simulink model "x280_canfd_loopback"  (R2024b)
settings: Solver=FixedStepDiscrete  StartTime=0.0  StopTime=inf  FixedStep=0.001  RelTol=1e-3
PreLoadFcn:
  | setupX280CANLibrary;
InitFcn:
  | setupX280CANLibrary;
libraries: x280_can_library x5, canfdmsglib x4
settings Model: Creator=Administrator  LastModifiedBy=Administrator
settings OptimizationCC: EnhancedBackFolding=on  PassReuseOutputArgsAs=Individual arguments  ZeroExternalMemoryAtStartup=off  ZeroInternalMemoryAtStartup=off  MaxStackSize=64  OptimizeBlockOrder=speed  DifferentSizesBufferReuse=on  OptimizationCustomize=off  EfficientTunableParamExpr=on
settings DebuggingCC: ParameterTunabilityLossMsg=error
settings HardwareCC: ProdBitPerLong=64  ProdHWDeviceType=Intel->x86-64 (Linux 64)
settings SFSimCC: MATLABDynamicMemAlloc=off
settings RTWCC: Description=Embedded Coder  SystemTargetFile=ert.tlc  HardwareBoard=SimRT  TLCOptions="-aInlineSetEventsForThisBaseRateFcn=TLC_FALSE -aSuppressMultiTaskScheduler=TLC_FALSE  -aRateBasedStepFcn=0"  TemplateMakefile=ert_default_tmf  Toolchain=X280 portable-linux-toolchain
settings CodeAppCC: ForceParamTrailComments=on  IgnoreCustomStorageClasses=off  OperatorAnnotations=on  SimulinkDataObjDesc=on  SFDataObjDesc=on  InsertBlockDesc=on
settings ERTTargetCC: ExtMode=on  ExtModeTransport=2  ExtModeStaticAlloc=on  ExtModeMexFile=ext_xcp  ExtModeIntrfLevel=Level2 - Open  InlinedParameterPlacement=Hierarchical

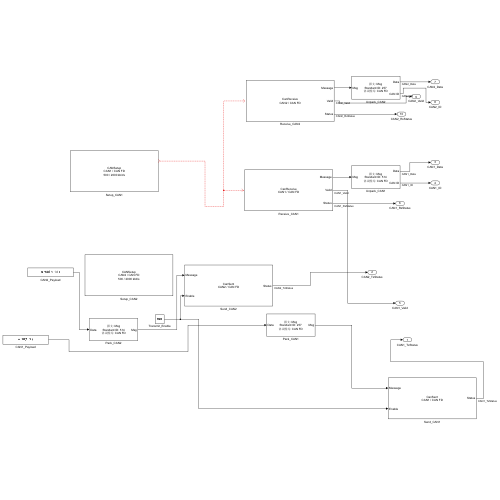
[thumbnail: Simulink's stored preview of the top-level diagram]
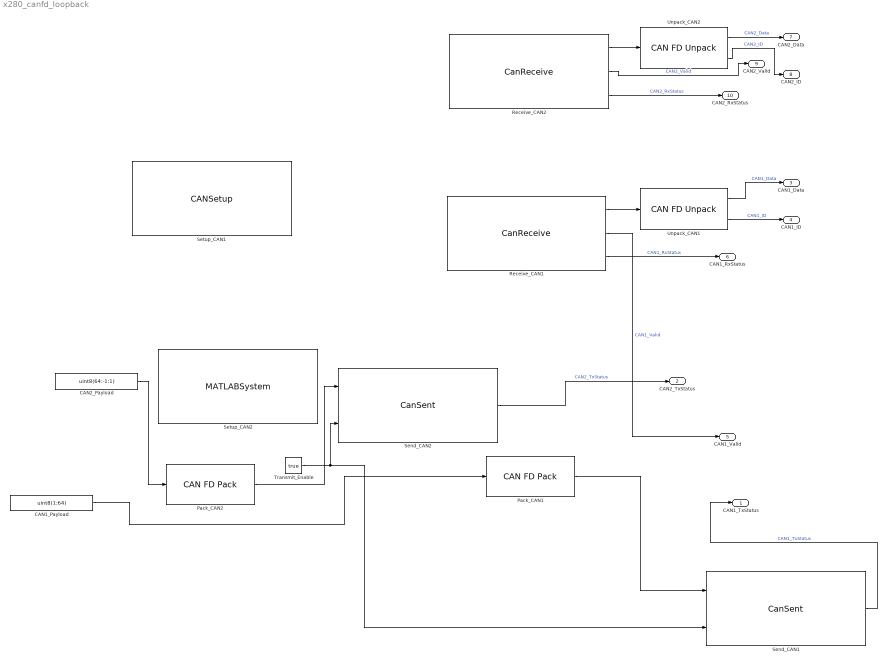
== system x280_canfd_loopback ==
  CAN1_Payload : Constant  Value=uint8(1:64)  SampleTime=0.001
  CAN2_Payload : Constant  Value=uint8(64:-1:1)  SampleTime=0.001
  Pack_CAN1 : canfdmsglib/CAN FD Pack  MsgList=(none)  MsgName=Msg  ProtocolMode=CAN FD  MsgIDType=Standard (11-bit identifier)  MsgIdentifier=257  CANIDInput=off  MsgLength=64  Remote=off  BRSSwitch=on  ApplyMinMax=off  SignalInfo={}
      settings: LibrarySourceBlock=canfdlib/CAN FD Pack  DataFormat=raw data
  Pack_CAN2 : canfdmsglib/CAN FD Pack  MsgList=(none)  MsgName=Msg  ProtocolMode=CAN FD  MsgIDType=Standard (11-bit identifier)  MsgIdentifier=514  CANIDInput=off  MsgLength=64  Remote=off  BRSSwitch=on  ApplyMinMax=off  SignalInfo={}
      settings: LibrarySourceBlock=canfdlib/CAN FD Pack  DataFormat=raw data
  Receive_CAN1 : x280_can_library/CanReceive  Priority=0  Channel=1  CANType=CAN FD  SampleTime=0.001
      settings: SourceProductName=X280 Linux TC1013 CAN
  Receive_CAN2 : x280_can_library/CanReceive  Priority=1  Channel=2  CANType=CAN FD  SampleTime=0.001
      settings: SourceProductName=X280 Linux TC1013 CAN
  Send_CAN1 : x280_can_library/CanSent  Priority=-50  Channel=1  CANType=CAN FD
      settings: SourceProductName=X280 Linux TC1013 CAN
  Send_CAN2 : x280_can_library/CanSent  Priority=-49  Channel=2  CANType=CAN FD
      settings: SourceProductName=X280 Linux TC1013 CAN
  Setup_CAN1 : x280_can_library/CANSetup  Priority=-100  Channel=1  CANType=CAN FD  BaudRate=500  DataBitRate=2000  Termination=true  DriverDirectory=/home/zh/.local/lib/tscan-thread-fix-20260926  SampleTime=0.001  HostTransport=Loopback
      settings: SourceProductName=X280 Linux TC1013 CAN
  Setup_CAN2 : MATLABSystem  Priority=-99  System=x280linux.can.CANSetup  Channel=2  CANType=CAN FD  BaudRate=500  DataBitRate=2000  Termination=true  DriverDirectory=/home/zh/.local/lib/tscan-thread-fix-20260926  SampleTime=0.001  HostTransport=Loopback
      mask Type: x280linux.can.CANSetup
      mask Display: disp(['CANSetup' char(10) 'CAN2 / CAN FD' char(10) '500 / 2000 kbit/s']);
  Transmit_Enable : Constant  Value=true  OutDataTypeStr=boolean  SampleTime=0.001
  Unpack_CAN1 : canfdmsglib/CAN FD Unpack  MsgList=(none)  MsgName=Msg  ProtocolMode=CAN FD  MsgIDType=Standard (11-bit identifier)  MsgIdentifier=514  MsgLength=64  SignalInfo={}  IDPort=on  TimestampPort=off  ErrorPort=off  RemotePort=off  LengthPort=off  StatusPort=off  BRSPort=off  ESIPort=off  DLCPort=off  ApplyMinMax=off
      settings: LibrarySourceBlock=canfdlib/CAN FD Unpack  DataFormat=raw data
  Unpack_CAN2 : canfdmsglib/CAN FD Unpack  MsgList=(none)  MsgName=Msg  ProtocolMode=CAN FD  MsgIDType=Standard (11-bit identifier)  MsgIdentifier=257  MsgLength=64  SignalInfo={}  IDPort=on  TimestampPort=off  ErrorPort=off  RemotePort=off  LengthPort=off  StatusPort=off  BRSPort=off  ESIPort=off  DLCPort=off  ApplyMinMax=off
      settings: LibrarySourceBlock=canfdlib/CAN FD Unpack  DataFormat=raw data
  CAN1_TxStatus : Outport
  CAN2_TxStatus : Outport  Port=2
  CAN1_Data : Outport  Port=3
  CAN1_ID : Outport  Port=4
  CAN1_Valid : Outport  Port=5
  CAN1_RxStatus : Outport  Port=6
  CAN2_Data : Outport  Port=7
  CAN2_ID : Outport  Port=8
  CAN2_Valid : Outport  Port=9
  CAN2_RxStatus : Outport  Port=10
  wires:
  ? -> ?
  Receive_CAN1/3 -> CAN1_RxStatus/1  "CAN1_RxStatus"
  Receive_CAN2/3 -> CAN2_RxStatus/1  "CAN2_RxStatus"
  Send_CAN2/1 -> CAN2_TxStatus/1  "CAN2_TxStatus"
  Pack_CAN2/1 -> Send_CAN2/1
  CAN2_Payload/1 -> Pack_CAN2/1
  CAN1_Payload/1 -> Pack_CAN1/1
  Unpack_CAN2/2 -> CAN2_ID/1  "CAN2_ID"
  Unpack_CAN1/2 -> CAN1_ID/1  "CAN1_ID"
  Pack_CAN1/1 -> Send_CAN1/1
  Receive_CAN1/1 -> Unpack_CAN1/1
  Unpack_CAN1/1 -> CAN1_Data/1  "CAN1_Data"
  Receive_CAN2/1 -> Unpack_CAN2/1
  Unpack_CAN2/1 -> CAN2_Data/1  "CAN2_Data"
  Transmit_Enable/1 -> Send_CAN2/2, Send_CAN1/2
  Send_CAN1/1 -> CAN1_TxStatus/1  "CAN1_TxStatus"
  Receive_CAN2/2 -> CAN2_Valid/1  "CAN2_Valid"
  Receive_CAN1/2 -> CAN1_Valid/1  "CAN1_Valid"
